simulink model "Evehicle"  (R2021a)
settings: Solver=VariableStepAuto  StartTime=0  StopTime=2474  RelTol=1e-3
undefined symbols (not defined in the file): sigbuilder_block
libraries: fl_lib x9, sdl_lib x6, nesl_utility x5, ee_lib x4, autolibshared x3
settings Model: Creator=rajes  LastModifiedBy=rajes
settings SolverCC: MaxConsecutiveMinStep=10

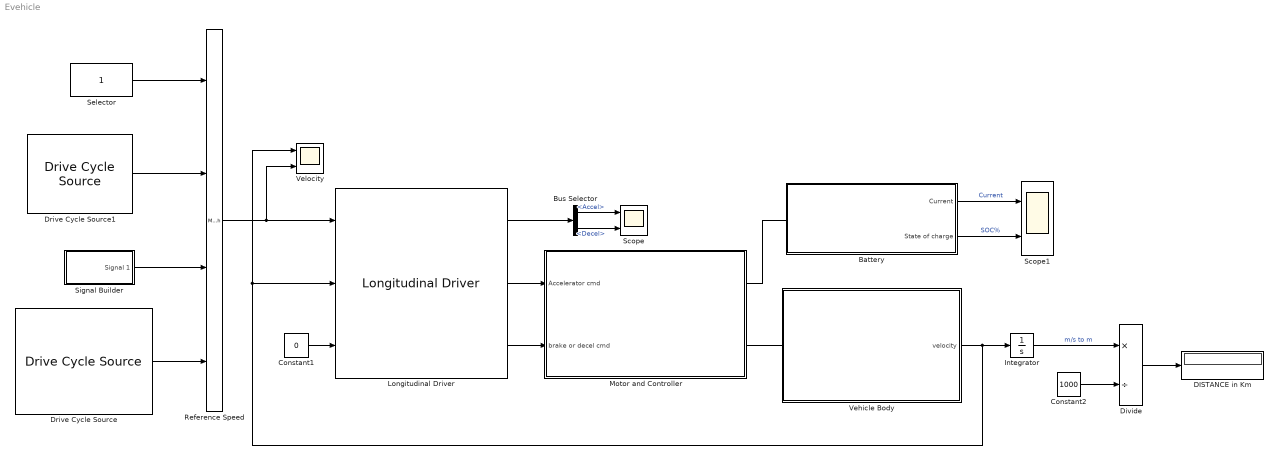
== system Evehicle ==
  "Battery " : Subsystem
  Bus Selector : BusSelector  OutputSignals=Accel,Decel
  Constant1 : Constant  Value=0
  Constant2 : Constant  Value=1000
  "DISTANCE in Km " : Display
  Divide : Product  Inputs=*/
  Drive Cycle Source : autolibshared/Drive Cycle Source  cycleVar=Artemis Motorway 150 kmph  fileVar=cycleFTP75.mat  tfinal="1068  seconds"  cycleRepeat=off  outAccPort=off  outGearPort=off  gearList=No gear data  t_wot1=5  xdot_woto=0  xdot_wot1=30  t_wot2=20  xdot_wot2=0  t_wotend=30  srcUnit=m/s  outUnit=m/s  srcAccUnit=m/s/s  outAccUnit=m/s^2  dt=0  aMode=1  faultOption=off  velBnd=2  velBndUnit=mph  inUnit=m/s  timeBnd=1  failOption=off  stopSim=off  maxFaultCnt=10  maxFaultTime=2  maxTotFaultTime=15  traceOption=off  dtTrace=1  traceWindow=10  lastDCname=FTP75  lastOutUnit=mph  lastDT=0  lastTB=1  lastSB=2  forceCalcBound=off
      settings: SourceProductBaseCode=PW,DR,MT,UV,VE
  Drive Cycle Source1 : autolibshared/Drive Cycle Source  cycleVar=FTP75  fileVar=cycleFTP75.mat  tfinal="2474  seconds"  cycleRepeat=off  outAccPort=off  outGearPort=off  gearList=No gear data  t_wot1=5  xdot_woto=0  xdot_wot1=30  t_wot2=60  xdot_wot2=0  t_wotend=100  srcUnit=m/s  outUnit=m/s  srcAccUnit=m/s/s  outAccUnit=m/s^2  dt=0  aMode=1  faultOption=off  velBnd=2  velBndUnit=mph  inUnit=m/s  timeBnd=1  failOption=off  stopSim=off  maxFaultCnt=10  maxFaultTime=2  maxTotFaultTime=15  traceOption=off  dtTrace=1  traceWindow=10  lastDCname=New York Bus Cycle  lastOutUnit=mph  lastDT=0  lastTB=1  lastSB=2  forceCalcBound=off
      settings: SourceProductBaseCode=PW,DR,MT,UV,VE
  Integrator : Integrator
  Longitudinal Driver : autolibshared/Longitudinal Driver  extAccelOvr=off  extDecelOvr=off  extAccelHld=off  extDecelHld=off  extAccelZero=off  extDecelZero=off  cntrlType=PI  shftType=None  velUnits=m/s  gearOut=off  Kp=20  Ki=1  Kff=0.1  Kg=0.1  VehVelVec=[0 100]  KffVec=[.1 .1]  KpVec=[10 10]  KiVec=[5 5]  KgVec=[0 0]  m=1500  Kpt=3000  tau=.1  L=2  aR=200  bR=2.5  cR=.5  g=9.81  vnom=5  Kaw=.1  tauerr=.03  tauPt=2  GearInit=0  tShift=.1  pdlVec=[0.1 0.4 0.5 0.9]  upShftTbl=[-1 12.9375 26.4375 39.9375 51.18749999999999 62.4375 72.84375 83.25;-1 16.3125 29.8125 43.3125 54.5624 65.8125 76.78125 87.75;-1 19.6875 33.1875 46.68749999999999 57.9375 69.1875 80.71875 92.25;-1 33 52.5 77.25 100.5 138.75 161.875 185]  dwnShftTbl=[1 9.5625 23.0625 36.5625 47.8125 59.0625 68.90625 78.75;1 12.9375 26.4375 39.9375 51.18749999999999 62.4375 72.84375 83.25;1 16.3125 29.8125 43.3125 54.562499 65.8125 76.78125 87.75;1 19.6875 33.1875 46.68749999999999 57.9375 69.1875 80.71875 92.25]  tClutch=.5  tRev=.5  tPark=120  aMode=1  UpGearVec="[0  1  2  3  4  5  6  7]"  DownGearVec="[1  2  3  4  5  6  7  8]"
      settings: SourceProductBaseCode=PW,DR,MT,UV,VE
  "Motor and Controller " : Subsystem
  "Reference Speed " : MultiPortSwitch
  Scope : Scope  NumInputPorts=2
  Scope1 : Scope  NumInputPorts=2
  "Selector " : Constant
  Signal Builder : Subsystem  Tag=STV Subsys  LoadFcn=sigbuilder_block('load');  StartFcn=sigbuilder_block('start');  StopFcn=sigbuilder_block('stop');  ClipboardFcn=sigbuilder_block('clipboard');  mask(Sigbuilder block){tuvar=[0:10]}
      mask help: Simulink:masks:SigbuilderBlock_MD
      mask init:
      | if ~strcmp(get_param(bdroot(gcbh),'SimulationStatus'),'stopped') tuvar = sigbuilder_block('maskInit'); end
      settings: CopyFcn=sigbuilder_block('copy');  DeleteFcn=sigbuilder_block('delete');  ModelCloseFcn=sigbuilder_block('modelClose');  PreSaveFcn=sigbuilder_block('preSave');  PauseFcn=sigbuilder_block('pause');  ContinueFcn=sigbuilder_block('continue');  NameChangeFcn=sigbuilder_block('namechange');  OpenFcn=sigbuilder_block('open',[389.4 121.2 550.8 400.2 ]);  CloseFcn=sigbuilder_block('close');
      mask Display: plot(0, 0, 100, 100,[2, 2, 32, 32, 2], [68, 8, 8, 68, 68],[32, 2], [38, 38], [32, 19, 2],[53, 60, 44], [32, 17, 17, 2],[16, 16, 31, 31]);txt = getActiveGroup(gcbh);text(2, 100, txt,'verticalAlignment', 'top');
  "Vehicle Body " : Subsystem
  "Velocity " : Scope  NumInputPorts=2
  wires:
  Bus Selector/1 -> Scope/1  "<Accel>"
  "Battery "/1(Current) -> Scope1/1  "Current"
  "Selector "/1 -> "Reference Speed "/1
  Longitudinal Driver/3 -> "Motor and Controller "/2(brake or decel cmd)
  Drive Cycle Source1/1 -> "Reference Speed "/2
  Longitudinal Driver/2 -> "Motor and Controller "/1(Accelerator cmd)
  "Vehicle Body "/1("velocity ") -> Integrator/1, Longitudinal Driver/2, "Velocity "/1
  Signal Builder/1(Signal 1) -> "Reference Speed "/3
  Constant1/1 -> Longitudinal Driver/3
  Divide/1 -> "DISTANCE in Km "/1
  "Reference Speed "/1 -> Longitudinal Driver/1, "Velocity "/2
  Longitudinal Driver/1 -> Bus Selector/1
  Bus Selector/2 -> Scope/2  "<Decel>"
  Integrator/1 -> Divide/1  "m/s to m"
  Constant2/1 -> Divide/2
  "Battery "/2("State of charge ") -> Scope1/2  "SOC%"
  Drive Cycle Source/1 -> "Reference Speed "/4
  connections:
  "Motor and Controller "/RConn1 -- "Battery "/LConn1
  "Vehicle Body "/LConn1 -- "Motor and Controller "/RConn2

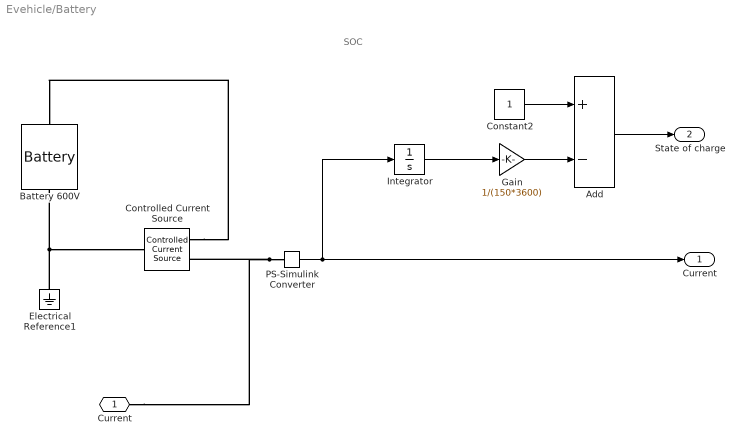
== system Evehicle/Battery  ==
  note: SOC
  Add : Sum  Inputs=+-
  Battery 600V : ee_lib/Sources/Battery  Vnom=600 V  prm_dir=1  R1_dis=2 Ohm  R1_ch=2 Ohm  R1=0.2 Ohm  prm_AH=1  AH=50 hr*A  V1=11.5 V  AH1=25 hr*A  prm_R2=1  R2=2000 Ohm  prm_dyn=1  Rp1=0.005 Ohm  tau1=30 s  Rp2=0.005 Ohm  tau2=30 s  Rp3=0.005 Ohm  tau3=30 s  Rp4=0.005 Ohm  tau4=30 s  Rp5=0.005 Ohm  tau5=30 s  prm_fade=1  N_fade=100  AH_fade=45 hr*A  R1_fade=2.02 Ohm  R1_ch_fade=2.02 Ohm  V1_fade=10.35 V  prm_age=1  prm_age_OCV=1  OCV_age=0.9  SOC_age=60  Tmeas_age=298.15 K  delta_time_age_vec=[0] d  temperature_age_vec=[273] K  OCV_scaling_age=2.2134e6  OCV_offset_age=1.632e6  temp_exp_age=0.515833569 V  t_exp_age=0.75  i_specify=off  i_priority=None  i=0 A  i_nominal_specify=off  i_nominal_unit=A  i_nominal_value=1  v_specify=off  v_priority=None  v=0 V  v_nominal_specify=off  v_nominal_unit=V  v_nominal_value=1  charge_specify=off  charge_priority=High  charge=50 hr*A  charge_nominal_specify=off  charge_nominal_unit=hr*A  charge_nominal_value=1  num_cycles_specify=off  num_cycles_priority=High  num_cycles=0  num_cycles_nominal_specify=off  num_cycles_nominal_unit=1  num_cycles_nominal_value=1  thermal_mass=30000 J/K  Tmeas=298.15 K  Vnom_T2=12 V  R1_T2=2.2 Ohm  R1_T2_dis=2.2 Ohm  R1_T2_ch=2.2 Ohm  V1_T2=11.4 V  R2_T2=2200 Ohm  Rp1_T2=0.005 Ohm  tau1_T2=30 s  Rp2_T2=0.005 Ohm  tau2_T2=30 s  Rp3_T2=0.005 Ohm  tau3_T2=30 s  Rp4_T2=0.005 Ohm  tau4_T2=30 s  Rp5_T2=0.005 Ohm  tau5_T2=30 s  Tmeas2=273.15 K  temperature_specify=off  temperature_priority=High  temperature=298.15 K  temperature_nominal_specify=off  temperature_nominal_unit=K  temperature_nominal_value=1
  Constant2 : Constant
  Controlled Current Source : fl_lib/Electrical/Electrical Sources/Controlled Current Source
  Electrical Reference1 : fl_lib/Electrical/Electrical Elements/Electrical Reference
  Gain : Gain  Gain=1/(150*3600)
  Integrator : Integrator
  PS-Simulink Converter : nesl_utility/PS-Simulink Converter  PhysicalDomain=network_engine_domain  SubClassName=ps_output  LeftPortType=input  RightPortType=output  PseudoPeriodic=off  Frequencies=[]  Unit=1  AffineConversion=off
      settings: SourceProductBaseCode=PW,SS
  "Current " : PMIOPort  Side=Left
  Current : Outport  VectorParamsAs1DForOutWhenUnconnected=off
  "State of charge " : Outport  Port=2  VectorParamsAs1DForOutWhenUnconnected=off
  wires:
  Add/1 -> "State of charge "/1
  Gain/1 -> Add/2
  Integrator/1 -> Gain/1
  PS-Simulink Converter/1 -> Current/1, Integrator/1
  Constant2/1 -> Add/1
  connections:
  Electrical Reference1/LConn1 -- Controlled Current Source/LConn1 -- Battery 600V/RConn1
  Controlled Current Source/RConn2 -- Battery 600V/LConn1
  PS-Simulink Converter/LConn1 -- "Current "/RConn1 -- Controlled Current Source/RConn1

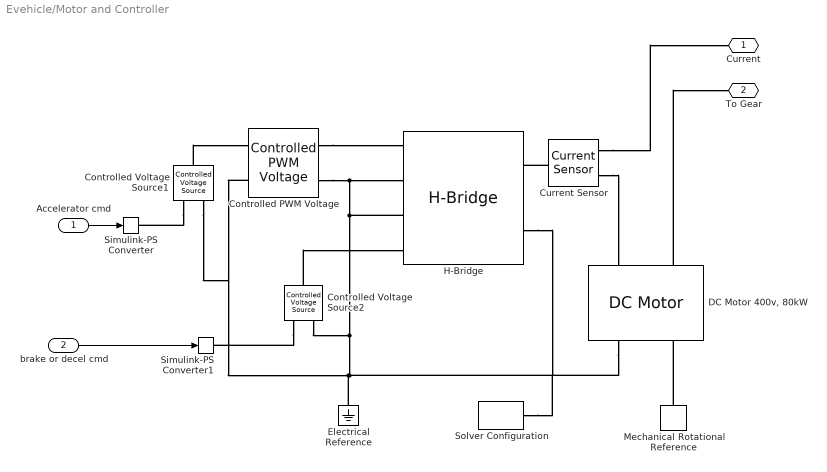
== system Evehicle/Motor and Controller  ==
  Accelerator cmd : Inport
  brake or decel cmd : Inport  Port=2
  Controlled PWM Voltage : ee_lib/Integrated Circuits/Controlled PWM Voltage  F=1000 Hz  TD=0 s  pulse_width_offset=0 s  pulse_min=0 s  Vmin=0 V  Vmax=5 V  Vm=400 V  pwm_or_av=2  event_type=1  sample_time=1e-6 s  u_min=0  u_max=1
  Controlled Voltage Source1 : fl_lib/Electrical/Electrical Sources/Controlled Voltage Source
  Controlled Voltage Source2 : fl_lib/Electrical/Electrical Sources/Controlled Voltage Source
  Current Sensor : fl_lib/Electrical/Electrical Sensors/Current Sensor
  "DC Motor 400v, 80kW" : ee_lib/Electromechanical/Brushed Motors/DC Motor  field_option=ee.enum.field_option.pm  Rf=100 Ohm  Lf=1 H  Laf=0.15 H  If0=0 A  parameterization=ee.enum.dcparam_option.load_speed  Ra=3.9 Ohm  La=12e-6 H  emf_or_torque=ee.enum.emf_or_torque.kv  Kv=0.072e-3 V/rpm  Ki=6.876e-4 N*m/A  T_stall=0.24e-3 N*m  w_max=6000 rpm  w_rated=4000 rpm  P_rated=80 kW  V_rated=400 V  J=0.01 g*cm^2  lam_param=ee.enum.lam_param.damping  lam=0 N*m/(rad/s)  i_noload=0 A  V_i_noload=1.5 V  speed0=0 rpm  enable_fault_armature=ee.enum.faults.faultEnable.no  rev_faulted=1 / 3  G_faulted_armature=1e-5 S  fault_trigger_armature=ee.enum.faults.faultTrigger.temporal  t_fault_armature=1 s  max_permissible_current_armature=inf A  t_fail_on_current_armature=1 s  enable_fault_field=ee.enum.faults.faultEnable.no  G_faulted_field=1e-5 S  fault_trigger_field=ee.enum.faults.faultTrigger.temporal  t_fault_field=1 s  max_permissible_current_field=inf A  t_fail_on_current_field=1 s  fault_action=ee.enum.faults.faultAction.none  alpha=3.93e-3 1/K  Tmeas=25 degC  thermal_mass=100 J/K  initial_temperature=25 degC
  Electrical Reference : fl_lib/Electrical/Electrical Elements/Electrical Reference
  H-Bridge : ee_lib/Semiconductors & Converters/Converters/H-Bridge  supply_ports=ee.enum.supply_ports.hidesupply  Venable=2.5 V  Vmax=5.0 V  Vreverse=2.5 V  Vbrake=2.5 V  Vm=400 V  pwm_or_av=2  regenerative_braking_mode=ee.enum.converters.regenerative_braking_mode.depends_on_rev  discontinuous=0  freewheeling_mode=1  Ron=0.1 Ohm  Don=0.05 Ohm  Goff=1e-6 S  Rload=10 Ohm  Lload=1e-5 H  F=10 kHz  thermal_mass=100 J/K  initial_temperature=298.15 K  Ron2=0.1 Ohm  Don2=0.05 Ohm  Tmeas=298.15 K  Tmeas2=398.15 K
  Mechanical Rotational Reference : fl_lib/Mechanical/Rotational Elements/Mechanical Rotational Reference
  Simulink-PS Converter : nesl_utility/Simulink-PS Converter  PhysicalDomain=network_engine_domain  SubClassName=ps_input  LeftPortType=input  RightPortType=output  PseudoPeriodic=off  Frequencies=[]  NoiseDistribution=none  NoiseParameters=[]  Unit=1  AffineConversion=off  FilteringAndDerivatives=provide  SimscapeFilterOrder=1  InputFilterTimeConstant=0.001  UdotUserProvided=0
      settings: SourceProductBaseCode=PW,SS
  Simulink-PS Converter1 : nesl_utility/Simulink-PS Converter  PhysicalDomain=network_engine_domain  SubClassName=ps_input  LeftPortType=input  RightPortType=output  PseudoPeriodic=off  Frequencies=[]  NoiseDistribution=none  NoiseParameters=[]  Unit=1  AffineConversion=off  FilteringAndDerivatives=provide  SimscapeFilterOrder=1  InputFilterTimeConstant=0.001  UdotUserProvided=0
      settings: SourceProductBaseCode=PW,SS
  Solver Configuration : nesl_utility/Solver Configuration  PhysicalDomain=network_engine_domain  SubClassName=solver  LeftPortType=input  RightPortType=generic  Tones=[]  Harmonics=[]  SimulateNoise=off  Profile=off  UseLocalSampling=off  EnableSwitchedLinearOptims=on  FrequencyDomain=off  UseCCode=off  RelTol=0.001  AbsTol=1e-06  MinStep=1e-09  ToWorkspace=off  RevertToSquareIcSolve=off  NumHomotopyIterations=100  PhasorMode=off  PhasorModeNumHarmonics=1  DoDC=off  ResidualTolerance=1e-09  UseLocalSolver=off  LocalSolverChoice=NE_BACKWARD_EULER_ADVANCER  LocalSolverSampleTime=0.001  DoFixedCost=off  MaxNonlinIter=3  MaxModeIter=2  ComputeImpulses=off  ImpulseIterations=2  LinearAlgebra=Full  EquationFormulation=NE_TIME_EF  DelaysMemoryBudget=1024  AutomaticFiltering=on  FilteringTimeConstant=0.001  PartitionStorageMethod=AS_NEEDED  PartitionMemoryBudget=1024  PartitionMethod=ROBUST
      settings: SourceProductBaseCode=PW,SS
  Current : PMIOPort  Side=Right
  "To Gear " : PMIOPort  Port=2  Side=Right
  wires:
  Accelerator cmd/1 -> Simulink-PS Converter/1
  brake or decel cmd/1 -> Simulink-PS Converter1/1
  connections:
  Controlled PWM Voltage/RConn2 -- Solver Configuration/RConn1 -- "DC Motor 400v, 80kW"/RConn1 -- H-Bridge/RConn2 -- Electrical Reference/LConn1 -- Controlled Voltage Source1/RConn2 -- Controlled PWM Voltage/LConn2 -- Controlled Voltage Source2/RConn2 -- H-Bridge/LConn3 -- H-Bridge/LConn2
  Current Sensor/RConn2 -- "DC Motor 400v, 80kW"/LConn1
  Controlled Voltage Source1/LConn1 -- Controlled PWM Voltage/LConn1
  Controlled Voltage Source2/LConn1 -- H-Bridge/LConn4
  Controlled PWM Voltage/RConn1 -- H-Bridge/LConn1
  Controlled Voltage Source1/RConn1 -- Simulink-PS Converter/RConn1
  Mechanical Rotational Reference/LConn1 -- "DC Motor 400v, 80kW"/RConn2
  Controlled Voltage Source2/RConn1 -- Simulink-PS Converter1/RConn1
  Current Sensor/LConn1 -- H-Bridge/RConn1
  Current Sensor/RConn1 -- Current/RConn1
  "DC Motor 400v, 80kW"/LConn2 -- "To Gear "/RConn1

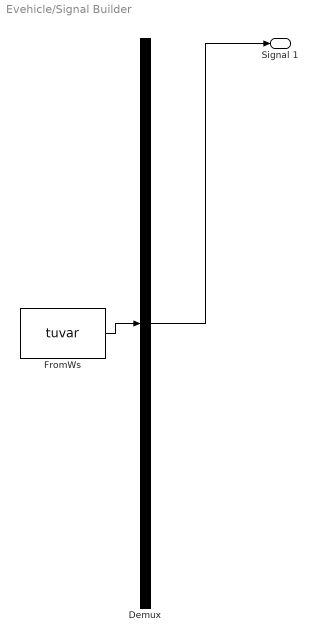
== system Evehicle/Signal Builder ==
  Demux : Demux  Tag=STV Demux  Outputs=1
      settings: DisplayOption=none
  FromWs : FromWorkspace  Tag=STV FromWs  VariableName=tuvar
      SigBuilderData=|
      | common.afterFinalStr = 'Extrapolate'
      | common.sampleTime = 0
      | dataSet.timeRange = [0 3600]
      | dataSet.name = 'Group 1'
      | sbobj.Groups.Name = 'Group 1'
      | sbobj.Groups.Signals.Name = 'Signal 1'
      | sbobj.Groups.Signals.XData = [0 4 4 3600]
      | sbobj.Groups.Signals.YData = [0 0 25 25]
      | sbobj.Groups.TimeRange = [0 3600]
  Signal 1 : Outport  Tag=STV Outport
  wires:
  Demux/1 -> Signal 1/1
  FromWs/1 -> Demux/1

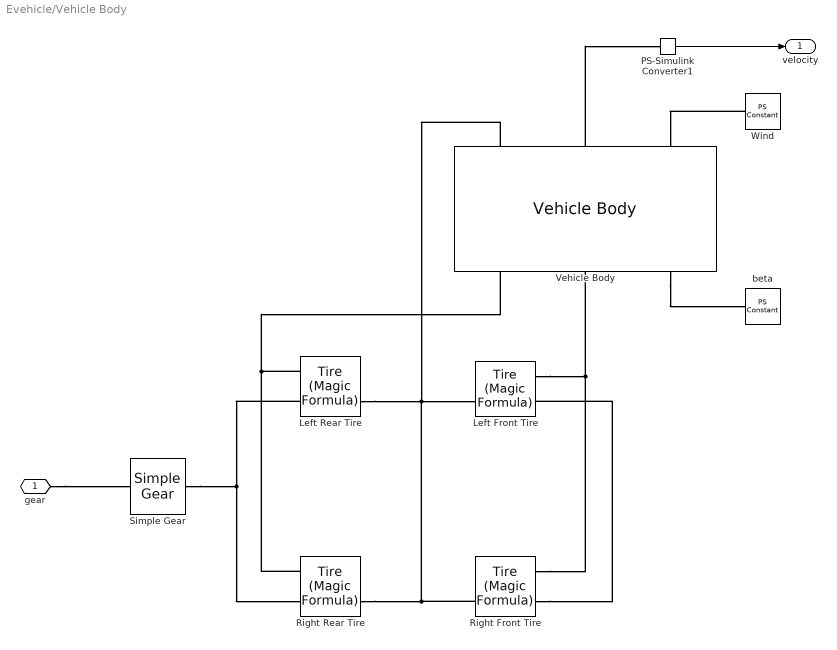
== system Evehicle/Vehicle Body  ==
  "Left Front Tire " : sdl_lib/Tires & Vehicles/Tire (Magic Formula)  parameterization=sdl.enum.magic_tire_model.peak  F_z1=3000 N  F_x1=3500 N  kappa1=10  B_m=10  C_m=1.9  D_m=1  E_m=0.97  fz0=4000 N  p_Cx=1.685  p_Dx=[1.21, -.037]  p_Ex=[.344, .095, -.02, 0]  p_Kx=[21.51, -.163, .245]  p_Hx=[-.002, .002]  p_Vx=[0, 0]  v_tr_thr=0.1 m/s  r_e=0.3 m  model_compliance=0  stiffness=1e6 N/m  damping=1000 N/(m/s)  model_inertia=0  inertia=1 kg*m^2  initial_velocity=0 rad/s  model_resistance=0  resistance_model=1  coeff=0.015  p_tire=250e3 Pa  alpha=-0.003  beta=0.97  coeff_a=84e-4  coeff_b=6.2e-4 s/m  coeff_c=1.6e-4 s^2/m^2  v_thr=0.001 m/s
  "Left Rear Tire " : sdl_lib/Tires & Vehicles/Tire (Magic Formula)  parameterization=sdl.enum.magic_tire_model.peak  F_z1=3000 N  F_x1=3500 N  kappa1=10  B_m=10  C_m=1.9  D_m=1  E_m=0.97  fz0=4000 N  p_Cx=1.685  p_Dx=[1.21, -.037]  p_Ex=[.344, .095, -.02, 0]  p_Kx=[21.51, -.163, .245]  p_Hx=[-.002, .002]  p_Vx=[0, 0]  v_tr_thr=0.1 m/s  r_e=0.3 m  model_compliance=0  stiffness=1e6 N/m  damping=1000 N/(m/s)  model_inertia=0  inertia=1 kg*m^2  initial_velocity=0 rad/s  model_resistance=0  resistance_model=1  coeff=0.015  p_tire=250e3 Pa  alpha=-0.003  beta=0.97  coeff_a=84e-4  coeff_b=6.2e-4 s/m  coeff_c=1.6e-4 s^2/m^2  v_thr=0.001 m/s
  PS-Simulink Converter1 : nesl_utility/PS-Simulink Converter  PhysicalDomain=network_engine_domain  SubClassName=ps_output  LeftPortType=input  RightPortType=output  PseudoPeriodic=off  Frequencies=[]  Unit=m/s  AffineConversion=on
      settings: SourceProductBaseCode=PW,SS
  "Right Front Tire " : sdl_lib/Tires & Vehicles/Tire (Magic Formula)  parameterization=sdl.enum.magic_tire_model.peak  F_z1=3000 N  F_x1=3500 N  kappa1=10  B_m=10  C_m=1.9  D_m=1  E_m=0.97  fz0=4000 N  p_Cx=1.685  p_Dx=[1.21, -.037]  p_Ex=[.344, .095, -.02, 0]  p_Kx=[21.51, -.163, .245]  p_Hx=[-.002, .002]  p_Vx=[0, 0]  v_tr_thr=0.1 m/s  r_e=0.3 m  model_compliance=0  stiffness=1e6 N/m  damping=1000 N/(m/s)  model_inertia=0  inertia=1 kg*m^2  initial_velocity=0 rad/s  model_resistance=0  resistance_model=1  coeff=0.015  p_tire=250e3 Pa  alpha=-0.003  beta=0.97  coeff_a=84e-4  coeff_b=6.2e-4 s/m  coeff_c=1.6e-4 s^2/m^2  v_thr=0.001 m/s
  Right Rear Tire : sdl_lib/Tires & Vehicles/Tire (Magic Formula)  parameterization=sdl.enum.magic_tire_model.peak  F_z1=3000 N  F_x1=3500 N  kappa1=10  B_m=10  C_m=1.9  D_m=1  E_m=0.97  fz0=4000 N  p_Cx=1.685  p_Dx=[1.21, -.037]  p_Ex=[.344, .095, -.02, 0]  p_Kx=[21.51, -.163, .245]  p_Hx=[-.002, .002]  p_Vx=[0, 0]  v_tr_thr=0.1 m/s  r_e=0.3 m  model_compliance=0  stiffness=1e6 N/m  damping=1000 N/(m/s)  model_inertia=0  inertia=1 kg*m^2  initial_velocity=0 rad/s  model_resistance=0  resistance_model=1  coeff=0.015  p_tire=250e3 Pa  alpha=-0.003  beta=0.97  coeff_a=84e-4  coeff_b=6.2e-4 s/m  coeff_c=1.6e-4 s^2/m^2  v_thr=0.001 m/s
  Simple Gear : sdl_lib/Gears/Simple Gear  ratio=2  rotation_direction=3-2*(1)  friction_model=sdl.enum.gear_efficiencies_load.off  mu_visc=[0, 0] N*m/(rad/s)  T_noload=0.1 N*m  T_nom=5 N*m  efficiency_nom=0.8  efficiency=0.8  temperature_TLU=[280, 300, 320] K  load_TLU=[1, 5, 10] N*m  efficiency_TLU=[.95, .9, .85]  efficiency_TLU2=[.85, .8, .75; .95, .9, .85; .85, .8, .7]  w_thr=0.01 rad/s  pwr_thr=0.001 W  thermal_mass=50 J/K  enable_faults=simscape.enum.onoff.off  efficiency_fault=0.05  external_fault=simscape.enum.onoff.off  temporal_fault=simscape.enum.onoff.off  fault_time=5 s  fault_angles=pi / 12 rad  report_fault=(1)-1  temperature_specify=off  temperature_priority=High  temperature=300 K  temperature_nominal_specify=off  temperature_nominal_unit=K  temperature_nominal_value=1
  Vehicle Body : sdl_lib/Tires & Vehicles/Vehicle Body  mass=1200 kg  n_w=2  x_f=1.4 m  x_r=1.6 m  y_c=0.5 m  mass_var=simscape.enum.onoff.off  model_pitch=simscape.enum.onoff.off  inertia=4000 kg*m^2  suspension_model=sdl.enum.linearTLU.linear  k_f=1e4 N/m  b_f=1e4 N/(m/s)  k_r=1e4 N/m  b_r=1e4 N/(m/s)  k_f_TLU=[-2000, -1000, 0, 1000, 2000] N  x_f_TLU=[-.4, -.2, 0, .2, .4] m  b_f_TLU=[-200, -100, 0, 100, 200] N  v_f_TLU=[-4, -2, 0, 2, 4] m/s  k_r_TLU=[-2000, -1000, 0, 1000, 2000] N  x_r_TLU=[-.4, -.2, 0, .2, .4] m  b_r_TLU=[-200, -100, 0, 100, 200] N  v_r_TLU=[-4, -2, 0, 2, 4] m/s  interp_method=simscape.enum.interpolation.linear  extrap_method=simscape.enum.extrapolation.linear  model_hardstop=simscape.enum.onoff.off  upper_bound_f=.25 m  lower_bound_f=-.25 m  stop_k_f=1e6 N/m  stop_b_f=150 N/(m/s)  upper_bound_r=.25 m  lower_bound_r=-.25 m  stop_k_r=1e6 N/m  stop_b_r=150 N/(m/s)  initial_pitch=0 rad  initial_pitch_rate=0 rad/s  g=9.81 m/s^2  liftoff_warning=simscape.enum.onoff.off  area=3 m^2  Cd=0.4  rho=1.18 kg/m^3  v_specify=on  v_priority=High  v=0 m/s  v_nominal_specify=off  v_nominal_unit=m/s  v_nominal_value=1
  Wind : fl_lib/Physical Signals/Sources/PS Constant  constant=0
  beta : fl_lib/Physical Signals/Sources/PS Constant  constant=0
  "gear " : PMIOPort  Side=Left
  "velocity " : Outport  Unit=m/s  VectorParamsAs1DForOutWhenUnconnected=off
  wires:
  PS-Simulink Converter1/1 -> "velocity "/1
  connections:
  Wind/RConn1 -- Vehicle Body/LConn3
  Vehicle Body/RConn3 -- beta/RConn1
  "Left Rear Tire "/LConn2 -- Right Rear Tire/LConn2 -- Simple Gear/RConn1
  "Left Rear Tire "/RConn2 -- Vehicle Body/LConn1 -- Right Rear Tire/RConn2 -- "Right Front Tire "/RConn2 -- "Left Front Tire "/RConn2
  Vehicle Body/LConn2 -- PS-Simulink Converter1/LConn1
  "gear "/RConn1 -- Simple Gear/LConn1
  "Right Front Tire "/LConn2 -- "Left Front Tire "/LConn2
  "Right Front Tire "/LConn1 -- Vehicle Body/RConn2 -- "Left Front Tire "/LConn1
  "Left Rear Tire "/LConn1 -- Right Rear Tire/LConn1 -- Vehicle Body/RConn1
